simulink model "mars_rover_terrain"  (R2025a)
settings: Solver=daessc  StartTime=0.0  StopTime=130*10  FixedStep=1e-10  MaxStep=1e-1  RelTol=1e-3  AbsTol=1e-3  EnableMultiTasking=on
undefined symbols (not defined in the file): arm_q0, Control, eeConfig, L1, L2, L3, LS1, LS3, R1, R2, R3, Rover, rover_path, RS1, RS3, X, Y, Z
libraries: sm_lib x137, nesl_utility x109, fl_lib x85, sdl_lib x20, ee_lib x10, mars_rover_lib x8, simulink x4, slpidlib x3, batteryecm_lib x2, robotcorelib x1, robotalgslib x1
(part 6 of 10)

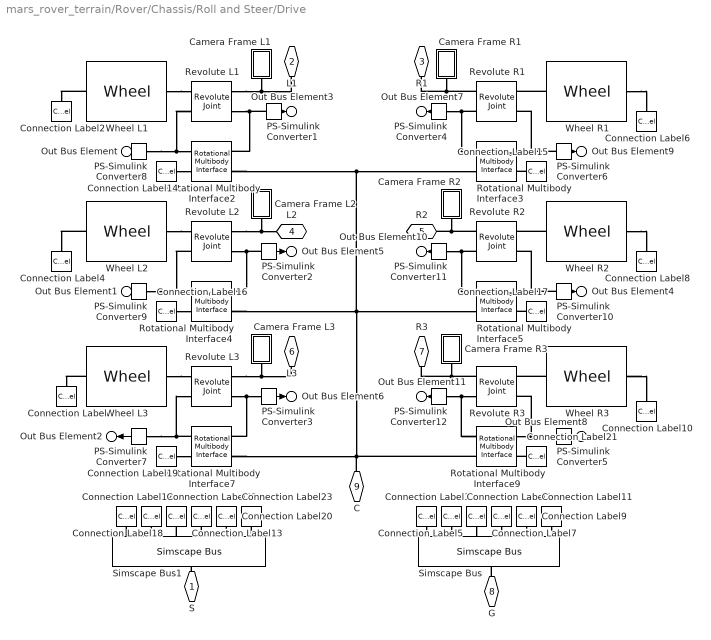
== system mars_rover_terrain/Rover/Chassis/Roll and Steer/Drive ==
  Camera Frame L1 : Subsystem
  Camera Frame L2 : Subsystem
  Camera Frame L3 : Subsystem
  Camera Frame R1 : Subsystem
  Camera Frame R2 : Subsystem
  Camera Frame R3 : Subsystem
  Connection Label : ConnectionLabel  Label=GL3
  Connection Label1 : ConnectionLabel  Label=GL3
  Connection Label10 : ConnectionLabel  Label=GR3
  Connection Label11 : ConnectionLabel  Label=GR3
  Connection Label12 : ConnectionLabel  Label=L1
  Connection Label13 : ConnectionLabel  Label=R1
  Connection Label14 : ConnectionLabel  Label=L1
  Connection Label15 : ConnectionLabel  Label=R1
  Connection Label16 : ConnectionLabel  Label=L2
  Connection Label17 : ConnectionLabel  Label=R2
  Connection Label18 : ConnectionLabel  Label=L2
  Connection Label19 : ConnectionLabel  Label=L3
  Connection Label2 : ConnectionLabel  Label=GL1
  Connection Label20 : ConnectionLabel  Label=R2
  Connection Label21 : ConnectionLabel  Label=R3
  Connection Label22 : ConnectionLabel  Label=L3
  Connection Label23 : ConnectionLabel  Label=R3
  Connection Label3 : ConnectionLabel  Label=GL1
  Connection Label4 : ConnectionLabel  Label=GL2
  Connection Label5 : ConnectionLabel  Label=GL2
  Connection Label6 : ConnectionLabel  Label=GR1
  Connection Label7 : ConnectionLabel  Label=GR1
  Connection Label8 : ConnectionLabel  Label=GR2
  Connection Label9 : ConnectionLabel  Label=GR2
  PS-Simulink Converter{1..12} (12 alike) : nesl_utility/PS-Simulink Converter  PhysicalDomain=network_engine_domain  SubClassName=ps_output  LeftPortType=input  RightPortType=output  PseudoPeriodic=off  Frequencies=[]  VectorFormat=1-D array  Unit=inherit  AffineConversion=off
  Revolute L1 : sm_lib/Joints/Revolute Joint  JointMode=Normal  CompositeWrenchDir=FollowerOnBase  CompositeWrenchFrame=BaseFrame  SenseConstraintForce=off  SenseConstraintTorque=off  SenseTotalForce=off  SenseTotalTorque=off  PositionTargetSpecify=off  PositionTargetPriority=High  PositionTargetValue=0  PositionTargetValueUnits=deg  VelocityTargetSpecify=off  VelocityTargetPriority=High  VelocityTargetValue=0  VelocityTargetValueUnits=deg/s  EquilibriumPosition=0  EquilibriumPositionUnits=deg  SpringStiffness=0  SpringStiffnessUnits=N*m/deg  DampingCoefficient=Rover.Drive.D  DampingCoefficientUnits=N*m/(deg/s)  LowerLimitSpecify=off  LowerLimitBound=-90  LowerLimitBoundUnits=deg  LowerLimitStiffness=1e4  LowerLimitStiffnessUnits=N*m/deg  LowerLimitDamping=10  LowerLimitDampingUnits=N*m/(deg/s)  LowerLimitTransitionRegionWidth=0.1  LowerLimitTransitionRegionWidthUnits=deg  UpperLimitSpecify=off  UpperLimitBound=90  UpperLimitBoundUnits=deg  UpperLimitStiffness=1e4  UpperLimitStiffnessUnits=N*m/deg  UpperLimitDamping=10  UpperLimitDampingUnits=N*m/(deg/s)  UpperLimitTransitionRegionWidth=0.1  UpperLimitTransitionRegionWidthUnits=deg  TorqueActuationMode=InputTorque  MotionActuationMode=ComputedMotion  SensePosition=off  SenseVelocity=on  SenseAcceleration=off  SenseTorqueForce=off  SenseLowerLimitTorqueForce=off  SenseUpperLimitTorqueForce=off
  Revolute L2 : sm_lib/Joints/Revolute Joint  JointMode=Normal  CompositeWrenchDir=FollowerOnBase  CompositeWrenchFrame=BaseFrame  SenseConstraintForce=off  SenseConstraintTorque=off  SenseTotalForce=off  SenseTotalTorque=off  PositionTargetSpecify=off  PositionTargetPriority=High  PositionTargetValue=0  PositionTargetValueUnits=deg  VelocityTargetSpecify=off  VelocityTargetPriority=High  VelocityTargetValue=0  VelocityTargetValueUnits=deg/s  EquilibriumPosition=0  EquilibriumPositionUnits=deg  SpringStiffness=0  SpringStiffnessUnits=N*m/deg  DampingCoefficient=Rover.Drive.D  DampingCoefficientUnits=N*m/(deg/s)  LowerLimitSpecify=off  LowerLimitBound=-90  LowerLimitBoundUnits=deg  LowerLimitStiffness=1e4  LowerLimitStiffnessUnits=N*m/deg  LowerLimitDamping=10  LowerLimitDampingUnits=N*m/(deg/s)  LowerLimitTransitionRegionWidth=0.1  LowerLimitTransitionRegionWidthUnits=deg  UpperLimitSpecify=off  UpperLimitBound=90  UpperLimitBoundUnits=deg  UpperLimitStiffness=1e4  UpperLimitStiffnessUnits=N*m/deg  UpperLimitDamping=10  UpperLimitDampingUnits=N*m/(deg/s)  UpperLimitTransitionRegionWidth=0.1  UpperLimitTransitionRegionWidthUnits=deg  TorqueActuationMode=InputTorque  MotionActuationMode=ComputedMotion  SensePosition=off  SenseVelocity=on  SenseAcceleration=off  SenseTorqueForce=off  SenseLowerLimitTorqueForce=off  SenseUpperLimitTorqueForce=off
  Revolute L3 : sm_lib/Joints/Revolute Joint  JointMode=Normal  CompositeWrenchDir=FollowerOnBase  CompositeWrenchFrame=BaseFrame  SenseConstraintForce=off  SenseConstraintTorque=off  SenseTotalForce=off  SenseTotalTorque=off  PositionTargetSpecify=off  PositionTargetPriority=High  PositionTargetValue=0  PositionTargetValueUnits=deg  VelocityTargetSpecify=off  VelocityTargetPriority=High  VelocityTargetValue=0  VelocityTargetValueUnits=deg/s  EquilibriumPosition=0  EquilibriumPositionUnits=deg  SpringStiffness=0  SpringStiffnessUnits=N*m/deg  DampingCoefficient=Rover.Drive.D  DampingCoefficientUnits=N*m/(deg/s)  LowerLimitSpecify=off  LowerLimitBound=-90  LowerLimitBoundUnits=deg  LowerLimitStiffness=1e4  LowerLimitStiffnessUnits=N*m/deg  LowerLimitDamping=10  LowerLimitDampingUnits=N*m/(deg/s)  LowerLimitTransitionRegionWidth=0.1  LowerLimitTransitionRegionWidthUnits=deg  UpperLimitSpecify=off  UpperLimitBound=90  UpperLimitBoundUnits=deg  UpperLimitStiffness=1e4  UpperLimitStiffnessUnits=N*m/deg  UpperLimitDamping=10  UpperLimitDampingUnits=N*m/(deg/s)  UpperLimitTransitionRegionWidth=0.1  UpperLimitTransitionRegionWidthUnits=deg  TorqueActuationMode=InputTorque  MotionActuationMode=ComputedMotion  SensePosition=off  SenseVelocity=on  SenseAcceleration=off  SenseTorqueForce=off  SenseLowerLimitTorqueForce=off  SenseUpperLimitTorqueForce=off
  Revolute R1 : sm_lib/Joints/Revolute Joint  JointMode=Normal  CompositeWrenchDir=FollowerOnBase  CompositeWrenchFrame=BaseFrame  SenseConstraintForce=off  SenseConstraintTorque=off  SenseTotalForce=off  SenseTotalTorque=off  PositionTargetSpecify=off  PositionTargetPriority=High  PositionTargetValue=0  PositionTargetValueUnits=deg  VelocityTargetSpecify=off  VelocityTargetPriority=High  VelocityTargetValue=0  VelocityTargetValueUnits=deg/s  EquilibriumPosition=0  EquilibriumPositionUnits=deg  SpringStiffness=0  SpringStiffnessUnits=N*m/deg  DampingCoefficient=Rover.Drive.D  DampingCoefficientUnits=N*m/(deg/s)  LowerLimitSpecify=off  LowerLimitBound=-90  LowerLimitBoundUnits=deg  LowerLimitStiffness=1e4  LowerLimitStiffnessUnits=N*m/deg  LowerLimitDamping=10  LowerLimitDampingUnits=N*m/(deg/s)  LowerLimitTransitionRegionWidth=0.1  LowerLimitTransitionRegionWidthUnits=deg  UpperLimitSpecify=off  UpperLimitBound=90  UpperLimitBoundUnits=deg  UpperLimitStiffness=1e4  UpperLimitStiffnessUnits=N*m/deg  UpperLimitDamping=10  UpperLimitDampingUnits=N*m/(deg/s)  UpperLimitTransitionRegionWidth=0.1  UpperLimitTransitionRegionWidthUnits=deg  TorqueActuationMode=InputTorque  MotionActuationMode=ComputedMotion  SensePosition=off  SenseVelocity=on  SenseAcceleration=off  SenseTorqueForce=off  SenseLowerLimitTorqueForce=off  SenseUpperLimitTorqueForce=off
  Revolute R2 : sm_lib/Joints/Revolute Joint  JointMode=Normal  CompositeWrenchDir=FollowerOnBase  CompositeWrenchFrame=BaseFrame  SenseConstraintForce=off  SenseConstraintTorque=off  SenseTotalForce=off  SenseTotalTorque=off  PositionTargetSpecify=off  PositionTargetPriority=High  PositionTargetValue=0  PositionTargetValueUnits=deg  VelocityTargetSpecify=off  VelocityTargetPriority=High  VelocityTargetValue=0  VelocityTargetValueUnits=deg/s  EquilibriumPosition=0  EquilibriumPositionUnits=deg  SpringStiffness=0  SpringStiffnessUnits=N*m/deg  DampingCoefficient=Rover.Drive.D  DampingCoefficientUnits=N*m/(deg/s)  LowerLimitSpecify=off  LowerLimitBound=-90  LowerLimitBoundUnits=deg  LowerLimitStiffness=1e4  LowerLimitStiffnessUnits=N*m/deg  LowerLimitDamping=10  LowerLimitDampingUnits=N*m/(deg/s)  LowerLimitTransitionRegionWidth=0.1  LowerLimitTransitionRegionWidthUnits=deg  UpperLimitSpecify=off  UpperLimitBound=90  UpperLimitBoundUnits=deg  UpperLimitStiffness=1e4  UpperLimitStiffnessUnits=N*m/deg  UpperLimitDamping=10  UpperLimitDampingUnits=N*m/(deg/s)  UpperLimitTransitionRegionWidth=0.1  UpperLimitTransitionRegionWidthUnits=deg  TorqueActuationMode=InputTorque  MotionActuationMode=ComputedMotion  SensePosition=off  SenseVelocity=on  SenseAcceleration=off  SenseTorqueForce=off  SenseLowerLimitTorqueForce=off  SenseUpperLimitTorqueForce=off
  Revolute R3 : sm_lib/Joints/Revolute Joint  JointMode=Normal  CompositeWrenchDir=FollowerOnBase  CompositeWrenchFrame=BaseFrame  SenseConstraintForce=off  SenseConstraintTorque=off  SenseTotalForce=off  SenseTotalTorque=off  PositionTargetSpecify=off  PositionTargetPriority=High  PositionTargetValue=0  PositionTargetValueUnits=deg  VelocityTargetSpecify=off  VelocityTargetPriority=High  VelocityTargetValue=0  VelocityTargetValueUnits=deg/s  EquilibriumPosition=0  EquilibriumPositionUnits=deg  SpringStiffness=0  SpringStiffnessUnits=N*m/deg  DampingCoefficient=Rover.Drive.D  DampingCoefficientUnits=N*m/(deg/s)  LowerLimitSpecify=off  LowerLimitBound=-90  LowerLimitBoundUnits=deg  LowerLimitStiffness=1e4  LowerLimitStiffnessUnits=N*m/deg  LowerLimitDamping=10  LowerLimitDampingUnits=N*m/(deg/s)  LowerLimitTransitionRegionWidth=0.1  LowerLimitTransitionRegionWidthUnits=deg  UpperLimitSpecify=off  UpperLimitBound=90  UpperLimitBoundUnits=deg  UpperLimitStiffness=1e4  UpperLimitStiffnessUnits=N*m/deg  UpperLimitDamping=10  UpperLimitDampingUnits=N*m/(deg/s)  UpperLimitTransitionRegionWidth=0.1  UpperLimitTransitionRegionWidthUnits=deg  TorqueActuationMode=InputTorque  MotionActuationMode=ComputedMotion  SensePosition=off  SenseVelocity=on  SenseAcceleration=off  SenseTorqueForce=off  SenseLowerLimitTorqueForce=off  SenseUpperLimitTorqueForce=off
  Rotational Multibody Interface{2..5,7,9} (6 alike) : fl_lib/Mechanical/Multibody Interfaces/Rotational Multibody Interface
  Simscape Bus : SimscapeBus  HierarchyStrings=L1;L2;L3;R1;R2;R3
  Simscape Bus1 : SimscapeBus  HierarchyStrings=L1;L2;L3;R1;R2;R3
  Wheel L1 : mars_rover_lib/Wheel  popup_leftRight=Left  pt_cld_loc=Rover.Wheel.wheel_point_cloud  pt_cld_rad=0.5  pt_cld_clr=[0.07451 0.6235 1]  pt_cld_opc=1
  Wheel L2 : mars_rover_lib/Wheel  popup_leftRight=Left  pt_cld_loc=Rover.Wheel.wheel_point_cloud  pt_cld_rad=0.5  pt_cld_clr=[0.07451 0.6235 1]  pt_cld_opc=1
  Wheel L3 : mars_rover_lib/Wheel  popup_leftRight=Left  pt_cld_loc=Rover.Wheel.wheel_point_cloud  pt_cld_rad=0.5  pt_cld_clr=[0.07451 0.6235 1]  pt_cld_opc=1
  Wheel R1 : mars_rover_lib/Wheel  popup_leftRight=Right  pt_cld_loc=Rover.Wheel.wheel_point_cloud  pt_cld_rad=0.5  pt_cld_clr=[0.07451 0.6235 1]  pt_cld_opc=1
  Wheel R2 : mars_rover_lib/Wheel  popup_leftRight=Right  pt_cld_loc=Rover.Wheel.wheel_point_cloud  pt_cld_rad=0.5  pt_cld_clr=[0.07451 0.6235 1]  pt_cld_opc=1
  Wheel R3 : mars_rover_lib/Wheel  popup_leftRight=Right  pt_cld_loc=Rover.Wheel.wheel_point_cloud  pt_cld_rad=0.5  pt_cld_clr=[0.07451 0.6235 1]  pt_cld_opc=1
  S : PMIOPort  Side=Left
  L1 : PMIOPort  Port=2  Side=Left
  R1 : PMIOPort  Port=3  Side=Right
  L2 : PMIOPort  Port=4  Side=Left
  R2 : PMIOPort  Port=5  Side=Right
  L3 : PMIOPort  Port=6  Side=Left
  R3 : PMIOPort  Port=7  Side=Right
  G : PMIOPort  Port=8  Side=Right
  C : PMIOPort  Port=9  Side=Left
  Out Bus Element : Outport  PortName=m  Element=w.L1
  Out Bus Element1 : Outport  PortName=m  Element=w.L2
  Out Bus Element2 : Outport  PortName=m  Element=w.L3
  Out Bus Element9 : Outport  PortName=m  Element=w.R1
  Out Bus Element4 : Outport  PortName=m  Element=w.R2
  Out Bus Element8 : Outport  PortName=m  Element=w.R3
  Out Bus Element3 : Outport  PortName=m  Element=trq.L1
  Out Bus Element5 : Outport  PortName=m  Element=trq.L2
  Out Bus Element6 : Outport  PortName=m  Element=trq.L3
  Out Bus Element7 : Outport  PortName=m  Element=trq.R1
  Out Bus Element10 : Outport  PortName=m  Element=trq.R2
  Out Bus Element11 : Outport  PortName=m  Element=trq.R3
  wires:
  PS-Simulink Converter7/1 -> Out Bus Element2/1
  PS-Simulink Converter5/1 -> Out Bus Element8/1
  PS-Simulink Converter9/1 -> Out Bus Element1/1
  PS-Simulink Converter6/1 -> Out Bus Element9/1
  PS-Simulink Converter8/1 -> Out Bus Element/1
  PS-Simulink Converter10/1 -> Out Bus Element4/1
  PS-Simulink Converter1/1 -> Out Bus Element3/1
  PS-Simulink Converter2/1 -> Out Bus Element5/1
  PS-Simulink Converter3/1 -> Out Bus Element6/1
  PS-Simulink Converter4/1 -> Out Bus Element7/1
  PS-Simulink Converter11/1 -> Out Bus Element10/1
  PS-Simulink Converter12/1 -> Out Bus Element11/1
  connections:
  Revolute L1/LConn2 -- PS-Simulink Converter1/LConn1 -- Rotational Multibody Interface2/LConn1
  Connection Label17/LConn1 -- Rotational Multibody Interface5/RConn2
  Wheel L2/RConn1 -- Revolute L2/RConn1
  Wheel L1/RConn1 -- Revolute L1/RConn1
  Connection Label3/LConn1 -- Simscape Bus/LConn1
  Rotational Multibody Interface7/RConn1 -- Revolute L3/RConn2 -- PS-Simulink Converter7/LConn1
  Connection Label9/LConn1 -- Simscape Bus/LConn5
  Wheel R3/LConn1 -- Connection Label10/LConn1
  Wheel R3/RConn1 -- Revolute R3/RConn1
  Revolute L2/RConn2 -- PS-Simulink Converter9/LConn1 -- Rotational Multibody Interface4/RConn1
  Rotational Multibody Interface3/RConn1 -- Revolute R1/RConn2 -- PS-Simulink Converter6/LConn1
  Rotational Multibody Interface4/LConn2 -- Rotational Multibody Interface7/LConn2 -- C/RConn1 -- Rotational Multibody Interface9/LConn2 -- Rotational Multibody Interface2/LConn2 -- Rotational Multibody Interface3/LConn2 -- Rotational Multibody Interface5/LConn2
  Connection Label1/LConn1 -- Simscape Bus/LConn3
  Revolute L1/RConn2 -- PS-Simulink Converter8/LConn1 -- Rotational Multibody Interface2/RConn1
  Connection Label5/LConn1 -- Simscape Bus/LConn2
  Wheel R1/LConn1 -- Connection Label6/LConn1
  Wheel R2/LConn1 -- Connection Label8/LConn1
  Revolute R1/LConn1 -- R1/RConn1 -- Camera Frame R1/LConn1
  Wheel L1/LConn1 -- Connection Label2/LConn1
  Rotational Multibody Interface9/RConn1 -- Revolute R3/RConn2 -- PS-Simulink Converter5/LConn1
  G/RConn1 -- Simscape Bus/RConn1
  Connection Label14/LConn1 -- Rotational Multibody Interface2/RConn2
  Wheel R2/RConn1 -- Revolute R2/RConn1
  Connection Label7/LConn1 -- Simscape Bus/LConn4
  Revolute L2/LConn1 -- Camera Frame L2/LConn1 -- L2/RConn1
  Wheel R1/RConn1 -- Revolute R1/RConn1
  Wheel L2/LConn1 -- Connection Label4/LConn1
  Connection Label15/LConn1 -- Rotational Multibody Interface3/RConn2
  Revolute R1/LConn2 -- Rotational Multibody Interface3/LConn1 -- PS-Simulink Converter4/LConn1
  Connection Label21/LConn1 -- Rotational Multibody Interface9/RConn2
  Wheel L3/RConn1 -- Revolute L3/RConn1
  Revolute L3/LConn2 -- PS-Simulink Converter3/LConn1 -- Rotational Multibody Interface7/LConn1
  Connection Label19/LConn1 -- Rotational Multibody Interface7/RConn2
  Rotational Multibody Interface5/RConn1 -- Revolute R2/RConn2 -- PS-Simulink Converter10/LConn1
  Revolute R2/LConn1 -- Camera Frame R2/LConn1 -- R2/RConn1
  Revolute L3/LConn1 -- Camera Frame L3/LConn1 -- L3/RConn1
  Rotational Multibody Interface9/LConn1 -- PS-Simulink Converter12/LConn1 -- Revolute R3/LConn2
  Revolute L1/LConn1 -- L1/RConn1 -- Camera Frame L1/LConn1
  Connection Label11/LConn1 -- Simscape Bus/LConn6
  Revolute L2/LConn2 -- PS-Simulink Converter2/LConn1 -- Rotational Multibody Interface4/LConn1
  Connection Label16/LConn1 -- Rotational Multibody Interface4/RConn2
  Wheel L3/LConn1 -- Connection Label/LConn1
  Revolute R2/LConn2 -- PS-Simulink Converter11/LConn1 -- Rotational Multibody Interface5/LConn1
  Revolute R3/LConn1 -- R3/RConn1 -- Camera Frame R3/LConn1
  Simscape Bus1/LConn1 -- Connection Label12/LConn1
  Simscape Bus1/LConn2 -- Connection Label18/LConn1
  Simscape Bus1/LConn3 -- Connection Label22/LConn1
  Simscape Bus1/LConn4 -- Connection Label13/LConn1
  Simscape Bus1/LConn5 -- Connection Label20/LConn1
  Simscape Bus1/LConn6 -- Connection Label23/LConn1
  S/RConn1 -- Simscape Bus1/RConn1

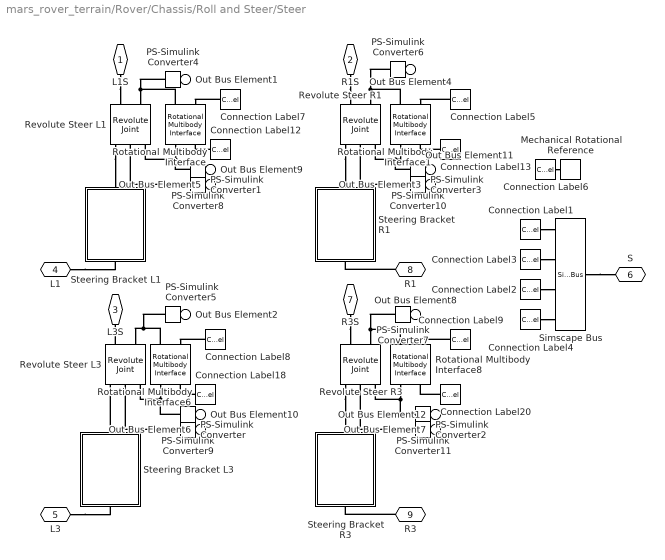
== system mars_rover_terrain/Rover/Chassis/Roll and Steer/Steer ==
  Connection Label1 : ConnectionLabel  Label=LS1
  Connection Label12 : ConnectionLabel  Label=LS1
  Connection Label13 : ConnectionLabel  Label=RS1
  Connection Label18 : ConnectionLabel  Label=LS3
  Connection Label2 : ConnectionLabel  Label=RS1
  Connection Label20 : ConnectionLabel  Label=RS3
  Connection Label3 : ConnectionLabel  Label=LS3
  Connection Label4 : ConnectionLabel  Label=RS3
  Connection Label{5..9} (5 alike) : ConnectionLabel  Label=C
  Mechanical Rotational Reference : fl_lib/Mechanical/Rotational Elements/Mechanical Rotational Reference
  PS-Simulink Converter{,1..3} (4 alike) : nesl_utility/PS-Simulink Converter  PhysicalDomain=network_engine_domain  SubClassName=ps_output  LeftPortType=input  RightPortType=output  PseudoPeriodic=off  Frequencies=[]  VectorFormat=1-D array  Unit=deg  AffineConversion=off
  PS-Simulink Converter{4..11} (8 alike) : nesl_utility/PS-Simulink Converter  PhysicalDomain=network_engine_domain  SubClassName=ps_output  LeftPortType=input  RightPortType=output  PseudoPeriodic=off  Frequencies=[]  VectorFormat=1-D array  Unit=inherit  AffineConversion=off
  Revolute Steer L1 : sm_lib/Joints/Revolute Joint  JointMode=Normal  CompositeWrenchDir=FollowerOnBase  CompositeWrenchFrame=BaseFrame  SenseConstraintForce=off  SenseConstraintTorque=off  SenseTotalForce=off  SenseTotalTorque=off  PositionTargetSpecify=on  PositionTargetPriority=High  PositionTargetValue=0  PositionTargetValueUnits=deg  VelocityTargetSpecify=off  VelocityTargetPriority=High  VelocityTargetValue=0  VelocityTargetValueUnits=deg/s  EquilibriumPosition=0  EquilibriumPositionUnits=deg  SpringStiffness=0  SpringStiffnessUnits=N*m/deg  DampingCoefficient=Rover.Steer.D  DampingCoefficientUnits=N*m/(deg/s)  LowerLimitSpecify=off  LowerLimitBound=-90  LowerLimitBoundUnits=deg  LowerLimitStiffness=1e4  LowerLimitStiffnessUnits=N*m/deg  LowerLimitDamping=10  LowerLimitDampingUnits=N*m/(deg/s)  LowerLimitTransitionRegionWidth=0.1  LowerLimitTransitionRegionWidthUnits=deg  UpperLimitSpecify=off  UpperLimitBound=90  UpperLimitBoundUnits=deg  UpperLimitStiffness=1e4  UpperLimitStiffnessUnits=N*m/deg  UpperLimitDamping=10  UpperLimitDampingUnits=N*m/(deg/s)  UpperLimitTransitionRegionWidth=0.1  UpperLimitTransitionRegionWidthUnits=deg  TorqueActuationMode=InputTorque  MotionActuationMode=ComputedMotion  SensePosition=on  SenseVelocity=on  SenseAcceleration=off  SenseTorqueForce=off  SenseLowerLimitTorqueForce=off  SenseUpperLimitTorqueForce=off
  Revolute Steer L3 : sm_lib/Joints/Revolute Joint  JointMode=Normal  CompositeWrenchDir=FollowerOnBase  CompositeWrenchFrame=BaseFrame  SenseConstraintForce=off  SenseConstraintTorque=off  SenseTotalForce=off  SenseTotalTorque=off  PositionTargetSpecify=on  PositionTargetPriority=High  PositionTargetValue=0  PositionTargetValueUnits=deg  VelocityTargetSpecify=off  VelocityTargetPriority=High  VelocityTargetValue=0  VelocityTargetValueUnits=deg/s  EquilibriumPosition=0  EquilibriumPositionUnits=deg  SpringStiffness=0  SpringStiffnessUnits=N*m/deg  DampingCoefficient=Rover.Steer.D  DampingCoefficientUnits=N*m/(deg/s)  LowerLimitSpecify=off  LowerLimitBound=-90  LowerLimitBoundUnits=deg  LowerLimitStiffness=1e4  LowerLimitStiffnessUnits=N*m/deg  LowerLimitDamping=10  LowerLimitDampingUnits=N*m/(deg/s)  LowerLimitTransitionRegionWidth=0.1  LowerLimitTransitionRegionWidthUnits=deg  UpperLimitSpecify=off  UpperLimitBound=90  UpperLimitBoundUnits=deg  UpperLimitStiffness=1e4  UpperLimitStiffnessUnits=N*m/deg  UpperLimitDamping=10  UpperLimitDampingUnits=N*m/(deg/s)  UpperLimitTransitionRegionWidth=0.1  UpperLimitTransitionRegionWidthUnits=deg  TorqueActuationMode=InputTorque  MotionActuationMode=ComputedMotion  SensePosition=on  SenseVelocity=on  SenseAcceleration=off  SenseTorqueForce=off  SenseLowerLimitTorqueForce=off  SenseUpperLimitTorqueForce=off
  Revolute Steer R1 : sm_lib/Joints/Revolute Joint  JointMode=Normal  CompositeWrenchDir=FollowerOnBase  CompositeWrenchFrame=BaseFrame  SenseConstraintForce=off  SenseConstraintTorque=off  SenseTotalForce=off  SenseTotalTorque=off  PositionTargetSpecify=on  PositionTargetPriority=High  PositionTargetValue=0  PositionTargetValueUnits=deg  VelocityTargetSpecify=off  VelocityTargetPriority=High  VelocityTargetValue=0  VelocityTargetValueUnits=deg/s  EquilibriumPosition=0  EquilibriumPositionUnits=deg  SpringStiffness=0  SpringStiffnessUnits=N*m/deg  DampingCoefficient=Rover.Steer.D  DampingCoefficientUnits=N*m/(deg/s)  LowerLimitSpecify=off  LowerLimitBound=-90  LowerLimitBoundUnits=deg  LowerLimitStiffness=1e4  LowerLimitStiffnessUnits=N*m/deg  LowerLimitDamping=10  LowerLimitDampingUnits=N*m/(deg/s)  LowerLimitTransitionRegionWidth=0.1  LowerLimitTransitionRegionWidthUnits=deg  UpperLimitSpecify=off  UpperLimitBound=90  UpperLimitBoundUnits=deg  UpperLimitStiffness=1e4  UpperLimitStiffnessUnits=N*m/deg  UpperLimitDamping=10  UpperLimitDampingUnits=N*m/(deg/s)  UpperLimitTransitionRegionWidth=0.1  UpperLimitTransitionRegionWidthUnits=deg  TorqueActuationMode=InputTorque  MotionActuationMode=ComputedMotion  SensePosition=on  SenseVelocity=on  SenseAcceleration=off  SenseTorqueForce=off  SenseLowerLimitTorqueForce=off  SenseUpperLimitTorqueForce=off
  Revolute Steer R3 : sm_lib/Joints/Revolute Joint  JointMode=Normal  CompositeWrenchDir=FollowerOnBase  CompositeWrenchFrame=BaseFrame  SenseConstraintForce=off  SenseConstraintTorque=off  SenseTotalForce=off  SenseTotalTorque=off  PositionTargetSpecify=on  PositionTargetPriority=High  PositionTargetValue=0  PositionTargetValueUnits=deg  VelocityTargetSpecify=off  VelocityTargetPriority=High  VelocityTargetValue=0  VelocityTargetValueUnits=deg/s  EquilibriumPosition=0  EquilibriumPositionUnits=deg  SpringStiffness=0  SpringStiffnessUnits=N*m/deg  DampingCoefficient=Rover.Steer.D  DampingCoefficientUnits=N*m/(deg/s)  LowerLimitSpecify=off  LowerLimitBound=-90  LowerLimitBoundUnits=deg  LowerLimitStiffness=1e4  LowerLimitStiffnessUnits=N*m/deg  LowerLimitDamping=10  LowerLimitDampingUnits=N*m/(deg/s)  LowerLimitTransitionRegionWidth=0.1  LowerLimitTransitionRegionWidthUnits=deg  UpperLimitSpecify=off  UpperLimitBound=90  UpperLimitBoundUnits=deg  UpperLimitStiffness=1e4  UpperLimitStiffnessUnits=N*m/deg  UpperLimitDamping=10  UpperLimitDampingUnits=N*m/(deg/s)  UpperLimitTransitionRegionWidth=0.1  UpperLimitTransitionRegionWidthUnits=deg  TorqueActuationMode=InputTorque  MotionActuationMode=ComputedMotion  SensePosition=on  SenseVelocity=on  SenseAcceleration=off  SenseTorqueForce=off  SenseLowerLimitTorqueForce=off  SenseUpperLimitTorqueForce=off
  Rotational Multibody Interface{,1,6,8} (4 alike) : fl_lib/Mechanical/Multibody Interfaces/Rotational Multibody Interface
  Simscape Bus : SimscapeBus  HierarchyStrings=LS1;LS3;RS1;RS3
  Steering Bracket L1 : Subsystem
      mask Display: image('mars_rover_terrain_chassis_steerbracketl.png');
  Steering Bracket L3 : Subsystem
      mask Display: image('mars_rover_terrain_chassis_steerbracketl.png');
  Steering Bracket R1 : Subsystem
      mask Display: image('mars_rover_terrain_chassis_steerbracketr.png');
  Steering Bracket R3 : Subsystem
      mask Display: image('mars_rover_terrain_chassis_steerbracketr.png');
  L1S : PMIOPort  Side=Left
  R1S : PMIOPort  Port=2  Side=Right
  L3S : PMIOPort  Port=3  Side=Left
  L1 : PMIOPort  Port=4  Side=Left
  L3 : PMIOPort  Port=5  Side=Left
  S : PMIOPort  Port=6  Side=Left
  R3S : PMIOPort  Port=7  Side=Right
  R1 : PMIOPort  Port=8  Side=Right
  R3 : PMIOPort  Port=9  Side=Right
  Out Bus Element5 : Outport  PortName=m  Element=q.L1
  Out Bus Element6 : Outport  PortName=m  Element=q.L3
  Out Bus Element3 : Outport  PortName=m  Element=q.R1
  Out Bus Element7 : Outport  PortName=m  Element=q.R3
  Out Bus Element2 : Outport  PortName=m  Element=trq.L3
  Out Bus Element1 : Outport  PortName=m  Element=trq.L1
  Out Bus Element4 : Outport  PortName=m  Element=trq.R1
  Out Bus Element8 : Outport  PortName=m  Element=trq.R3
  Out Bus Element9 : Outport  PortName=m  Element=w.L1
  Out Bus Element10 : Outport  PortName=m  Element=w.L3
  Out Bus Element11 : Outport  PortName=m  Element=w.R1
  Out Bus Element12 : Outport  PortName=m  Element=w.R3
  wires:
  PS-Simulink Converter3/1 -> Out Bus Element3/1
  PS-Simulink Converter1/1 -> Out Bus Element5/1
  PS-Simulink Converter/1 -> Out Bus Element6/1
  PS-Simulink Converter2/1 -> Out Bus Element7/1
  PS-Simulink Converter4/1 -> Out Bus Element1/1
  PS-Simulink Converter5/1 -> Out Bus Element2/1
  PS-Simulink Converter6/1 -> Out Bus Element4/1
  PS-Simulink Converter7/1 -> Out Bus Element8/1
  PS-Simulink Converter8/1 -> Out Bus Element9/1
  PS-Simulink Converter9/1 -> Out Bus Element10/1
  PS-Simulink Converter10/1 -> Out Bus Element11/1
  PS-Simulink Converter11/1 -> Out Bus Element12/1
  connections:
  Rotational Multibody Interface1/RConn1 -- Revolute Steer R1/RConn3 -- PS-Simulink Converter10/LConn1
  Rotational Multibody Interface1/LConn1 -- PS-Simulink Converter6/LConn1 -- Revolute Steer R1/LConn2
  Rotational Multibody Interface/LConn1 -- PS-Simulink Converter4/LConn1 -- Revolute Steer L1/LConn2
  Connection Label8/LConn1 -- Rotational Multibody Interface6/LConn2
  Revolute Steer R1/RConn1 -- Steering Bracket R1/RConn1
  Connection Label18/LConn1 -- Rotational Multibody Interface6/RConn2
  Connection Label7/LConn1 -- Rotational Multibody Interface/LConn2
  Connection Label9/LConn1 -- Rotational Multibody Interface8/LConn2
  Steering Bracket L3/LConn1 -- Revolute Steer L3/RConn1
  Revolute Steer R3/RConn1 -- Steering Bracket R3/RConn1
  Connection Label5/LConn1 -- Rotational Multibody Interface1/LConn2
  L1S/RConn1 -- Revolute Steer L1/LConn1
  Rotational Multibody Interface/RConn1 -- Revolute Steer L1/RConn3 -- PS-Simulink Converter8/LConn1
  Rotational Multibody Interface8/RConn1 -- Revolute Steer R3/RConn3 -- PS-Simulink Converter11/LConn1
  Revolute Steer L1/RConn1 -- Steering Bracket L1/LConn1
  Connection Label13/LConn1 -- Rotational Multibody Interface1/RConn2
  R3S/RConn1 -- Revolute Steer R3/LConn1
  Rotational Multibody Interface6/LConn1 -- PS-Simulink Converter5/LConn1 -- Revolute Steer L3/LConn2
  Revolute Steer L3/LConn1 -- L3S/RConn1
  R1/RConn1 -- Steering Bracket R1/LConn1
  Connection Label20/LConn1 -- Rotational Multibody Interface8/RConn2
  R3/RConn1 -- Steering Bracket R3/LConn1
  Rotational Multibody Interface8/LConn1 -- PS-Simulink Converter7/LConn1 -- Revolute Steer R3/LConn2
  R1S/RConn1 -- Revolute Steer R1/LConn1
  Rotational Multibody Interface6/RConn1 -- Revolute Steer L3/RConn3 -- PS-Simulink Converter9/LConn1
  Connection Label12/LConn1 -- Rotational Multibody Interface/RConn2
  L1/RConn1 -- Steering Bracket L1/RConn1
  L3/RConn1 -- Steering Bracket L3/RConn1
  Connection Label1/LConn1 -- Simscape Bus/LConn1
  Connection Label3/LConn1 -- Simscape Bus/LConn2
  Connection Label2/LConn1 -- Simscape Bus/LConn3
  Connection Label4/LConn1 -- Simscape Bus/LConn4
  Simscape Bus/RConn1 -- S/RConn1
  PS-Simulink Converter1/LConn1 -- Revolute Steer L1/RConn2
  PS-Simulink Converter3/LConn1 -- Revolute Steer R1/RConn2
  PS-Simulink Converter/LConn1 -- Revolute Steer L3/RConn2
  PS-Simulink Converter2/LConn1 -- Revolute Steer R3/RConn2
  Connection Label6/LConn1 -- Mechanical Rotational Reference/LConn1

== system mars_rover_terrain/Control/Arm Control/ Trajectory Planner/SampleDropOffCmdLogic/Enabled Subsystem1 ==
  In1 : Inport
  Enable : EnablePort
  Out1 : Outport
  wires:
  In1/1 -> Out1/1

== system mars_rover_terrain/Control/Arm Control/ Trajectory Planner/SampleLoc wrt arm base/Enabled Subsystem1 ==
  In1 : Inport
  Enable : EnablePort
  Out1 : Outport
  wires:
  In1/1 -> Out1/1

== system mars_rover_terrain/Control/Arm Control/ Trajectory Planner/SamplePickUpCmdLogic/Enabled Subsystem1 ==
  In1 : Inport
  Enable : EnablePort
  Out1 : Outport
  wires:
  In1/1 -> Out1/1

== system mars_rover_terrain/Control/Chassis Control/Target Direction and Speed/hold/RoverStopTime ==
  Enable : Inport
  Clock : Clock
  Constant2 : Constant
  Enabled Subsystem1 : Subsystem  TreatAsAtomicUnit=on
      settings: MinAlgLoopOccurrences=on
  Switch : Switch  Criteria=u2 > Threshold  SaturateOnIntegerOverflow=off  InputSameDT=off
  Unit Delay : UnitDelay  SampleTime=-1  HasFrameUpgradeWarning=on
  DeAccelTime : Outport
  wires:
  Enabled Subsystem1/1(Out1) -> Switch/2
  Enable/1 -> Enabled Subsystem1/Enable
  Switch/1 -> Unit Delay/1
  Unit Delay/1 -> DeAccelTime/1, Switch/1
  Clock/1 -> Switch/3
  Constant2/1 -> Enabled Subsystem1/1(In1)
